simulink model "flightControlSystem"  (R2026b)
settings: Solver=ode3  StopTime=TFinal
PreLoadFcn:
  | InitVars;
  | definePX4ParamsBus;
undefined symbols (not defined in the file): control_power, DiscIntNeverNeededParam, init, MC_PITCHRATE_MAX, MC_ROLLRATE_MAX, MC_YAWRATE_MAX, PX4_Params_Default, SampleTime, timestamp
libraries: px4Utilslib x52, px4uORBlib x10, vrlib x8, aerolibutil x8, simulink x5, sharedutil x3, matrix_library x2, raspberrypiutilitieslib x2, px4Peripheralslib x2, sharedtransform x1, px4Sensorslib x1
(part 1 of 4)
settings Model: SimulationMode=external  Creator=The MathWorks, Inc.  LastModifiedBy=vishn
settings SolverCC: AutoInsertRateTranBlk=on  PositivePriorityOrder=on
settings DataIOCC: InputTimeTolerance=on
settings OptimizationCC: DifferentSizesBufferReuse=on  EfficientTunableParamExpr=on  EnhancedBackFolding=on  MaxStackSize=64  OptimizationCustomize=off  OptimizeBlockOrder=speed  PassReuseOutputArgsAs=Individual arguments  RemoveInternalMemoryZeroInit=on  RemoveRootLevelIOMemoryZeroInit=on
settings DebuggingCC: MultiTaskDSMMsg=none  ParameterPrecisionLossMsg=none  ParameterTunabilityLossMsg=error
settings HardwareCC: ProdHWDeviceType=ARM Compatible->ARM Cortex  ProdLargestAtomicFloat=Double  ProdLargestAtomicInteger=Long  ProdLongLongMode=on
settings SFSimCC: MATLABDynamicMemAlloc=off  SimTargetLang=C++
settings RTWCC: Description=Embedded Coder  HardwareBoard=PX4 Pixhawk 6c  SystemTargetFile=ert.tlc  TLCOptions="-aInlineSetEventsForThisBaseRateFcn=TLC_FALSE -aSuppressMultiTaskScheduler=TLC_FALSE  -aRateBasedStepFcn=0"  TargetLang=C++  TemplateMakefile=ert_default_tmf  Toolchain=GNU Tools for PX4 Autopilots
settings CodeAppCC: ForceParamTrailComments=on  IgnoreCustomStorageClasses=off  InsertBlockDesc=on  OperatorAnnotations=on  SFDataObjDesc=on  SimulinkDataObjDesc=on
settings ERTTargetCC: ExtModeIntrfLevel=Level2 - Open  ExtModeMexFile=ext_xcp  ExtModeStaticAlloc=on  SupportVariableSizeSignals=on

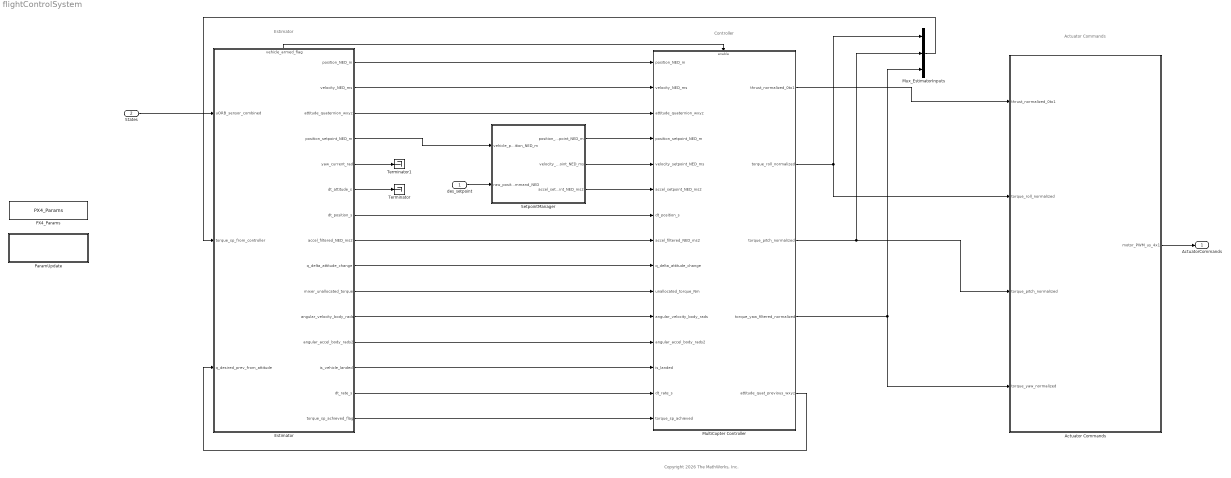
== system flightControlSystem ==
  note: Actuator Commands
  note: Estimator
  note: Controller
  note: Copyright 2026 The MathWorks, Inc.
  des_setpoint : Inport  OutDataTypeStr=Bus: desiredTargetSetpoints
  States : Inport  Port=2  OutDataTypeStr=Bus: UAVStatesBus
  Actuator Commands : Subsystem  Variant=on
  Estimator : Subsystem  Variant=on
      settings: PortSchema="{\"entries\":[{\"content\":{\"sides\":[{\"content\":{\"connectorIds\":[\"In1\",\"In2\",\"In3\"]},\"type\":\"ConnectorPlacement.EquallySpacedRectSide\",\"uuid\":\"982d90d8-ff1f-4cb9-8e33-8baf717922ad\"},{\"content\":{\"connectorIds\":[\"Out1\",\"Out2\",\"Out3\",\"Out4\",\"Out5\",\"Out6\",\"Out7\",\"Out8\",\"Out9\",\"Out10\",\"Out11\",\"Out12\",\"Out13\",\"Out14\",\"Out15\"],\"side\":\"RIGHT\"},\"type\":\"ConnectorPlacement.EquallySpacedRectSide\",\"uuid\":\"20bc02a1-8188-433b-a626-e8822f00966c\"},{\"content\":{\"connectorIds\":[\"Out16\"],\"side\":\"TOP\"},\"type\":\"ConnectorPlacement.EquallySpacedRectSide\",\"uuid\":\"edaeaf83-210e-410d-8d39-7cda3629118d\"}]},\"type\":\"ConnectorPlacement.EquallySpacedConnector\",\"uuid\":\"c0d6638f-6096-4882-ba89-b56950bc4adf\"}],\"packageUris\":[\"http://schema.mathworks.com/mf0/Connector/R2020b\"],\"version\":\"1.0\"}"
  MultiCopter Controller : Subsystem
  Mux_EstimatorInputs : Mux  Inputs=3
  PX4_Params : DataStoreMemory  DataStoreName=PX4_Params  WriteAfterWriteMsg=warning  InitialValue=PX4_Params_Default  ShowAdditionalParam=off  OutDataTypeStr=Bus: PX4_Params_Bus
  ParamUpdate : Subsystem  TreatAsAtomicUnit=on  Variant=on
  SetpointManager : Subsystem  Variant=on
  Terminator : Terminator
  Terminator1 : Terminator
  ActuatorCommands : Outport  OutDataTypeStr=Bus: setPWMInput
  wires:
  MultiCopter Controller/2(torque_roll_normalized) -> Actuator Commands/2(torque_roll_normalized), Mux_EstimatorInputs/1
  MultiCopter Controller/1(thrust_normalized_0to1) -> Actuator Commands/1(thrust_normalized_0to1)
  Estimator/11(angular_velocity_body_rads) -> MultiCopter Controller/11(angular_velocity_body_rads)
  MultiCopter Controller/4(torque_yaw_filtered_normalized) -> Mux_EstimatorInputs/3, Actuator Commands/4(torque_yaw_normalized)
  Estimator/3(attitude_quaternion_wxyz) -> MultiCopter Controller/3(attitude_quaternion_wxyz)
  MultiCopter Controller/5(attitude_quat_previous_wxyz) -> Estimator/3(q_desired_prev_from_attitude)
  SetpointManager/3(accel_setpoint_NED_ms2) -> MultiCopter Controller/6(accel_setpoint_NED_ms2)
  MultiCopter Controller/3(torque_pitch_normalized) -> Actuator Commands/3(torque_pitch_normalized), Mux_EstimatorInputs/2
  Estimator/10(mixer_unallocated_torque) -> MultiCopter Controller/10(unallocated_torque_Nm)
  Estimator/12(angular_accel_body_rads2) -> MultiCopter Controller/12(angular_accel_body_rads2)
  Mux_EstimatorInputs/1 -> Estimator/2(torque_sp_from_controller)
  Estimator/7(dt_position_s) -> MultiCopter Controller/7(dt_position_s)
  SetpointManager/1(position_setpoint_NED_m) -> MultiCopter Controller/4(position_setpoint_NED_m)
  Estimator/2(velocity_NED_ms) -> MultiCopter Controller/2(velocity_NED_ms)
  Estimator/8(accel_filtered_NED_ms2) -> MultiCopter Controller/8(accel_filtered_NED_ms2)
  Estimator/5(yaw_current_rad) -> Terminator1/1
  Estimator/6(dt_attitude_s) -> Terminator/1
  States/1 -> Estimator/1(uORB_sensor_combined)
  Actuator Commands/1(motor_PWM_us_4x1) -> ActuatorCommands/1
  Estimator/13(is_vehicle_landed) -> MultiCopter Controller/13(is_landed)
  SetpointManager/2(velocity_setpoint_NED_ms) -> MultiCopter Controller/5(velocity_setpoint_NED_ms)
  Estimator/4(position_setpoint_NED_m) -> SetpointManager/1(vehicle_position_NED_m)
  Estimator/1(position_NED_m) -> MultiCopter Controller/1(position_NED_m)
  Estimator/9(q_delta_attitude_change) -> MultiCopter Controller/9(q_delta_attitude_change)
  Estimator/16(vehicle_armed_flag) -> MultiCopter Controller/Enable
  Estimator/14(dt_rate_s) -> MultiCopter Controller/14(dt_rate_s)
  Estimator/15(torque_sp_achieved_flag) -> MultiCopter Controller/15(torque_sp_achieved)
  des_setpoint/1 -> SetpointManager/2(raw_position_command_NED)

== system flightControlSystem/Actuator Commands ==
  note: Simulation = true:
      | The subsystem processes the tau and thrust signals, computes the multicopter mixers, and generates the PWM signals required by the plant for closed-loop simulation.
      |
      | Simulation = false:
      | The subsystem processes the tau and thrust signals output from the controller and publishes them to the Torque and Thrust block. The PX4 mixer then computes the required outputs based on the selected multicopter configuration for flight operations.
  thrust_normalized_0to1 : Inport
  torque_roll_normalized : Inport  Port=2
  torque_pitch_normalized : Inport  Port=3
  torque_yaw_normalized : Inport  Port=4
  Actuator Commands : Subsystem  VariantControl=Simulation == false
  Simulation Actuator Commands : Subsystem  VariantControl=Simulation == true
  motor_PWM_us_4x1 : Outport

== system flightControlSystem/Estimator ==
  note: Simulation = true:
      | The subsystem provides the required estimator values from the 6-DoF Dynamics feedback for closed-loop simulation with the controller.
      |
      | Simulation = false:
      | The subsystem reads the required PX4 estimator values for the flight controller from the uOrb block.
  uORB_sensor_combined : Inport
  torque_sp_from_controller : Inport  Port=2
  q_desired_prev_from_attitude : Inport  Port=3
  Estimator : Subsystem  VariantControl=Simulation == false
  Simulation Estimator : Subsystem  VariantControl=Simulation == true
  position_NED_m : Outport
  velocity_NED_ms : Outport  Port=2
  attitude_quaternion_wxyz : Outport  Port=3
  position_setpoint_NED_m : Outport  Port=4
  yaw_current_rad : Outport  Port=5
  dt_attitude_s : Outport  Port=6
  dt_position_s : Outport  Port=7
  accel_filtered_NED_ms2 : Outport  Port=8
  q_delta_attitude_change : Outport  Port=9
  mixer_unallocated_torque : Outport  Port=10
  angular_velocity_body_rads : Outport  Port=11
  angular_accel_body_rads2 : Outport  Port=12
  is_vehicle_landed : Outport  Port=13
  dt_rate_s : Outport  Port=14
  torque_sp_achieved_flag : Outport  Port=15
  vehicle_armed_flag : Outport  Port=16

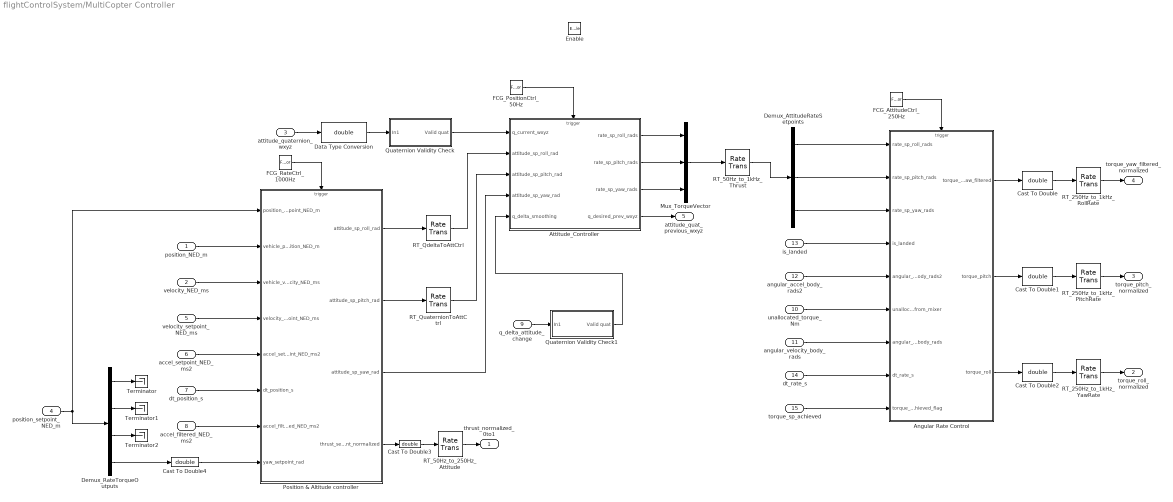
== system flightControlSystem/MultiCopter Controller ==
  position_NED_m : Inport
  velocity_NED_ms : Inport  Port=2
  attitude_quaternion_wxyz : Inport  Port=3
  position_setpoint_NED_m : Inport  Port=4
  velocity_setpoint_NED_ms : Inport  Port=5
  accel_setpoint_NED_ms2 : Inport  Port=6
  dt_position_s : Inport  Port=7
  accel_filtered_NED_ms2 : Inport  Port=8
  q_delta_attitude_change : Inport  Port=9
  unallocated_torque_Nm : Inport  Port=10
  angular_velocity_body_rads : Inport  Port=11
  angular_accel_body_rads2 : Inport  Port=12
  is_landed : Inport  Port=13
  dt_rate_s : Inport  Port=14
  torque_sp_achieved : Inport  Port=15
  Enable : EnablePort
  Angular Rate Control : Subsystem
  Attitude_Controller : Subsystem
  Cast To Double{,1..4} (5 alike) : DataTypeConversion  OutDataTypeStr=double  SaturateOnIntegerOverflow=off  RndMeth=Floor
  Data Type Conversion : DataTypeConversion  OutDataTypeStr=double  SaturateOnIntegerOverflow=off  RndMeth=Floor
  Demux_AttitudeRateSetpoints : Demux  Outputs=3
  Demux_RateTorqueOutputs : Demux
  FCG_AttitudeCtrl_250Hz : FunctionCallGenerator  SampleTime=0.001
  FCG_PositionCtrl_50Hz : FunctionCallGenerator  SampleTime=0.004
  FCG_RateCtrl_1000Hz : FunctionCallGenerator  SampleTime=0.02
  Mux_TorqueVector : Mux  Inputs=3
  Position & Altitude controller : Subsystem
  Quaternion Validity Check : Subsystem
  Quaternion Validity Check1 : Subsystem
  RT_250Hz_to_1kHz_PitchRate : RateTransition  OutPortSampleTime=SampleTime
  RT_250Hz_to_1kHz_RollRate : RateTransition  OutPortSampleTime=SampleTime
  RT_250Hz_to_1kHz_YawRate : RateTransition  OutPortSampleTime=SampleTime
  RT_50Hz_to_1kHz_Thrust : RateTransition
  RT_50Hz_to_250Hz_Attitude : RateTransition  OutPortSampleTime=SampleTime
  RT_QdeltaToAttCtrl : RateTransition
  RT_QuaternionToAttCtrl : RateTransition
  Terminator : Terminator
  Terminator1 : Terminator
  Terminator2 : Terminator
  thrust_normalized_0to1 : Outport
  torque_roll_normalized : Outport  Port=2
  torque_pitch_normalized : Outport  Port=3
  torque_yaw_filtered_normalized : Outport  Port=4
  attitude_quat_previous_wxyz : Outport  Port=5
  wires:
  unallocated_torque_Nm/1 -> Angular Rate Control/6(unallocated_torque_from_mixer)
  Demux_RateTorqueOutputs/4 -> Cast To Double4/1
  Demux_RateTorqueOutputs/2 -> Terminator1/1
  Demux_RateTorqueOutputs/3 -> Terminator2/1
  Data Type Conversion/1 -> Quaternion Validity Check/1(In1)
  attitude_quaternion_wxyz/1 -> Data Type Conversion/1
  Quaternion Validity Check/1(Valid quat) -> Attitude_Controller/1(q_current_wxyz)
  position_setpoint_NED_m/1 -> Position & Altitude controller/1(position_setpoint_NED_m), Demux_RateTorqueOutputs/1
  Demux_RateTorqueOutputs/1 -> Terminator/1
  q_delta_attitude_change/1 -> Quaternion Validity Check1/1(In1)
  FCG_RateCtrl_1000Hz/1 -> Position & Altitude controller/Trigger
  Attitude_Controller/4(q_desired_prev_wxyz) -> attitude_quat_previous_wxyz/1
  position_NED_m/1 -> Position & Altitude controller/2(vehicle_position_NED_m)
  dt_rate_s/1 -> Angular Rate Control/8(dt_rate_s)
  velocity_NED_ms/1 -> Position & Altitude controller/3(vehicle_velocity_NED_ms)
  angular_accel_body_rads2/1 -> Angular Rate Control/5(angular_accel_body_rads2)
  velocity_setpoint_NED_ms/1 -> Position & Altitude controller/4(velocity_setpoint_NED_ms)
  RT_250Hz_to_1kHz_YawRate/1 -> torque_roll_normalized/1
  Angular Rate Control/3(torque_roll) -> Cast To Double2/1
  Cast To Double4/1 -> Position & Altitude controller/8(yaw_setpoint_rad)
  accel_setpoint_NED_ms2/1 -> Position & Altitude controller/5(accel_setpoint_NED_ms2)
  dt_position_s/1 -> Position & Altitude controller/6(dt_position_s)
  RT_250Hz_to_1kHz_RollRate/1 -> torque_yaw_filtered_normalized/1
  Quaternion Validity Check1/1(Valid quat) -> Attitude_Controller/5(q_delta_smoothing)
  accel_filtered_NED_ms2/1 -> Position & Altitude controller/7(accel_filtered_NED_ms2)
  Position & Altitude controller/2(attitude_sp_pitch_rad) -> RT_QuaternionToAttCtrl/1
  Position & Altitude controller/3(attitude_sp_yaw_rad) -> Attitude_Controller/4(attitude_sp_yaw_rad)
  Position & Altitude controller/1(attitude_sp_roll_rad) -> RT_QdeltaToAttCtrl/1
  Position & Altitude controller/4(thrust_setpoint_normalized) -> Cast To Double3/1
  FCG_PositionCtrl_50Hz/1 -> Attitude_Controller/Trigger
  RT_QdeltaToAttCtrl/1 -> Attitude_Controller/2(attitude_sp_roll_rad)
  RT_QuaternionToAttCtrl/1 -> Attitude_Controller/3(attitude_sp_pitch_rad)
  Cast To Double3/1 -> RT_50Hz_to_250Hz_Attitude/1
  RT_50Hz_to_1kHz_Thrust/1 -> Demux_AttitudeRateSetpoints/1
  is_landed/1 -> Angular Rate Control/4(is_landed)
  RT_50Hz_to_250Hz_Attitude/1 -> thrust_normalized_0to1/1
  Mux_TorqueVector/1 -> RT_50Hz_to_1kHz_Thrust/1
  FCG_AttitudeCtrl_250Hz/1 -> Angular Rate Control/Trigger
  RT_250Hz_to_1kHz_PitchRate/1 -> torque_pitch_normalized/1
  angular_velocity_body_rads/1 -> Angular Rate Control/7(angular_velocity_body_rads)
  torque_sp_achieved/1 -> Angular Rate Control/9(torque_sp_achieved_flag)
  Angular Rate Control/1(torque_yaw_filtered) -> Cast To Double/1
  Angular Rate Control/2(torque_pitch) -> Cast To Double1/1
  Cast To Double1/1 -> RT_250Hz_to_1kHz_PitchRate/1
  Cast To Double/1 -> RT_250Hz_to_1kHz_RollRate/1
  Cast To Double2/1 -> RT_250Hz_to_1kHz_YawRate/1
  Attitude_Controller/1(rate_sp_roll_rads) -> Mux_TorqueVector/1
  Attitude_Controller/2(rate_sp_pitch_rads) -> Mux_TorqueVector/2
  Attitude_Controller/3(rate_sp_yaw_rads) -> Mux_TorqueVector/3
  Demux_AttitudeRateSetpoints/1 -> Angular Rate Control/1(rate_sp_roll_rads)
  Demux_AttitudeRateSetpoints/2 -> Angular Rate Control/2(rate_sp_pitch_rads)
  Demux_AttitudeRateSetpoints/3 -> Angular Rate Control/3(rate_sp_yaw_rads)

== system flightControlSystem/ParamUpdate ==
  note: 1) Add Subsystem or Model blocks as valid variant choices.
      | 2) You cannot connect blocks at this level. At simulation, connectivity is automatically
      | determined, based on the active variant and port name matching.
  HW_ParamUpdate : Subsystem  VariantControl=Simulation == false
  SimParamUpdate : Subsystem  VariantControl=Simulation == true

== system flightControlSystem/SetpointManager ==
  note: Simulation = true:
      | The subsystem forwards the target setpoint signal from the PerceptionGuidance block as a bus signal for controller processing.
      |
      | Simulation = false:
      | The subsystem reads the target setpoint values from the Serial Read block and makes them available to the flight controller.
  vehicle_position_NED_m : Inport
  raw_position_command_NED : Inport  Port=2
  Set target Position : Subsystem  VariantControl=Simulation == false
  Simulation Set target Position : Subsystem  VariantControl=Simulation == true
  position_setpoint_NED_m : Outport
  velocity_setpoint_NED_ms : Outport  Port=2
  accel_setpoint_NED_ms2 : Outport  Port=3

== system flightControlSystem/Actuator Commands/Actuator Commands ==
  thrust_normalized_0to1 : Inport
  torque_pitch_normalized : Inport  Port=2
  torque_roll_normalized : Inport  Port=3
  torque_yaw_normalized : Inport  Port=4
  Bus Creator1 : BusCreator  Inputs=8  OutDataTypeStr=Bus: setPWMInput
  Demux2 : Demux  Outputs=8
  MATLAB Function : MATLAB Function  TreatAsAtomicUnit=on
  "Using PX4 Mixers " : Subsystem  VariantControl=isUsingSimulinkMixer==false
  motor_PWM_us_4x1 : Outport
  wires:
  MATLAB Function/1(y) -> Demux2/1
  thrust_normalized_0to1/1 -> "Using PX4 Mixers "/1(tau_Thrust)
  torque_pitch_normalized/1 -> "Using PX4 Mixers "/2(tau_Pitch)
  torque_roll_normalized/1 -> "Using PX4 Mixers "/3(tau_Roll)
  Demux2/7 -> Bus Creator1/7  "M7"
  Demux2/5 -> Bus Creator1/5  "M5"
  Demux2/1 -> Bus Creator1/1  "M1"
  Demux2/3 -> Bus Creator1/3  "M3"
  Demux2/8 -> Bus Creator1/8  "M8"
  Demux2/6 -> Bus Creator1/6  "M6"
  Demux2/4 -> Bus Creator1/4  "M4"
  Demux2/2 -> Bus Creator1/2  "M2"
  torque_yaw_normalized/1 -> "Using PX4 Mixers "/4(tau_yaw)
  Bus Creator1/1 -> motor_PWM_us_4x1/1

== system flightControlSystem/Actuator Commands/Simulation Actuator Commands ==
  thrust_normalized_0to1 : Inport
  torque_pitch_normalized : Inport  Port=2
  torque_roll_normalized : Inport  Port=3
  torque_yaw_normalized : Inport  Port=4
  Mixer : Subsystem
  motor_PWM_us_4x1 : Outport
  wires:
  thrust_normalized_0to1/1 -> Mixer/1(tau_Thrust)
  Mixer/1(PWM_Input) -> motor_PWM_us_4x1/1
  torque_yaw_normalized/1 -> Mixer/2(tau_yaw)
  torque_pitch_normalized/1 -> Mixer/3(tau_Pitch)
  torque_roll_normalized/1 -> Mixer/4(tau_Roll)

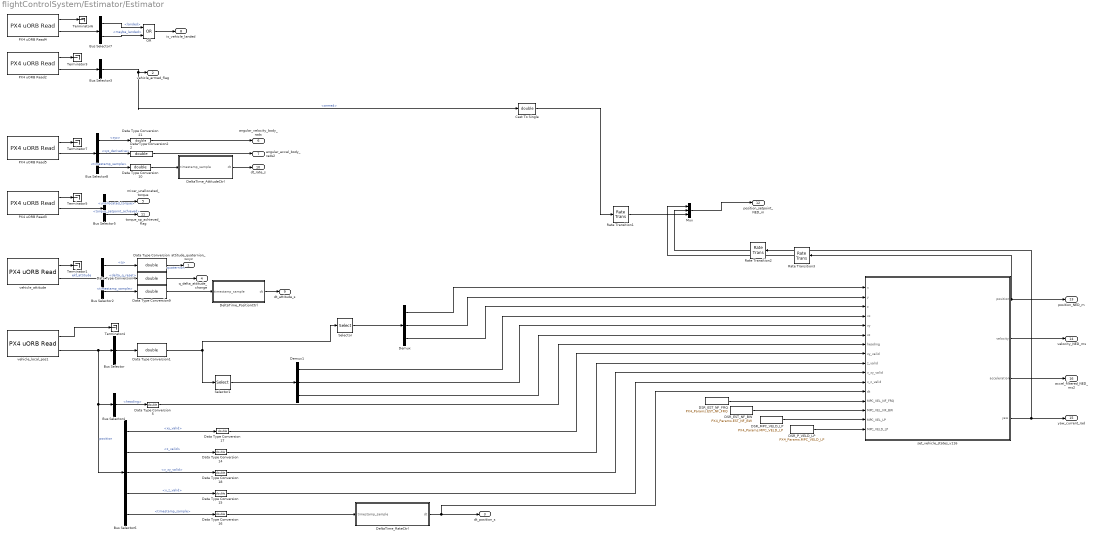
== system flightControlSystem/Estimator/Estimator ==
  Bus Selector : BusSelector  OutputSignals=x,y,z,vx,vy,vz,heading  OutputAsBus=on
  Bus Selector2 : BusSelector  OutputSignals=q,delta_q_reset,timestamp_sample
  Bus Selector3 : BusSelector  OutputSignals=armed
  Bus Selector4 : BusSelector  OutputSignals=heading
  Bus Selector5 : BusSelector  OutputSignals=unallocated_torque,torque_setpoint_achieved
  Bus Selector6 : BusSelector  OutputSignals=xy_valid,z_valid,v_xy_valid,v_z_valid,timestamp_sample
  Bus Selector7 : BusSelector  OutputSignals=landed,maybe_landed
  Bus Selector8 : BusSelector  OutputSignals=xyz,xyz_derivative,timestamp_sample
  Cast To Single : DataTypeConversion  OutDataTypeStr=double  SaturateOnIntegerOverflow=off  RndMeth=Floor
  DSR_EST_NF_BW : DataStoreRead  DataStoreName=PX4_Params  DataStoreElements=PX4_Params.EST_NF_BW  IndexOptions=Index vector (dialog)  Indices=1  OutputSizes=1
  DSR_EST_NF_FRQ : DataStoreRead  DataStoreName=PX4_Params  DataStoreElements=PX4_Params.EST_NF_FRQ  IndexOptions=Index vector (dialog)  Indices=1  OutputSizes=1
  DSR_MPC_VELD_LP : DataStoreRead  DataStoreName=PX4_Params  DataStoreElements=PX4_Params.MPC_VELD_LP  IndexOptions=Index vector (dialog)  Indices=1  OutputSizes=1
  DSR_P_VELD_LP : DataStoreRead  DataStoreName=PX4_Params  DataStoreElements=PX4_Params.MPC_VELD_LP  IndexOptions=Index vector (dialog)  Indices=1  OutputSizes=1
  Data Type Conversion{,1,4..5,9..10,14..18,21..22} (13 alike) : DataTypeConversion  OutDataTypeStr=double  SaturateOnIntegerOverflow=off  RndMeth=Floor
  DeltaTime_AttitudeCtrl : MATLAB Function  TreatAsAtomicUnit=on
  DeltaTime_PositionCtrl : MATLAB Function  TreatAsAtomicUnit=on
  DeltaTime_RateCtrl : MATLAB Function  TreatAsAtomicUnit=on
  Demux : Demux  Outputs=3
  Demux1 : Demux  Outputs=3
  Mux : Mux  Inputs=3
  OR : Logic  Operator=OR  IconShape=distinctive  AllPortsSameDT=off  OutDataTypeStr=boolean
  PX4 uORB Read2 : px4uORBlib/PX4 uORB Read  uORBMsg=ActuatorArmed  uORBTopicName=actuator_armed  SubscribeNonZeroInstance=off  selectInstanceNum=1  SampleTime=-1  isSingleTopicMsg=on  BlockingMode=off  BlockTimeout=1e-3
  PX4 uORB Read3 : px4uORBlib/PX4 uORB Read  uORBMsg=ControlAllocatorStatus  uORBTopicName=control_allocator_status  SubscribeNonZeroInstance=off  selectInstanceNum=1  SampleTime=-1  isSingleTopicMsg=on  BlockingMode=off  BlockTimeout=1e-3
  PX4 uORB Read4 : px4uORBlib/PX4 uORB Read  uORBMsg=VehicleLandDetected  uORBTopicName=vehicle_land_detected  SubscribeNonZeroInstance=off  selectInstanceNum=1  SampleTime=-1  isSingleTopicMsg=on  BlockingMode=off  BlockTimeout=1e-3
  PX4 uORB Read5 : px4uORBlib/PX4 uORB Read  uORBMsg=VehicleAngularVelocity  uORBTopicName=vehicle_angular_velocity  SubscribeNonZeroInstance=off  selectInstanceNum=1  SampleTime=-1  isSingleTopicMsg=off  BlockingMode=off  BlockTimeout=1e-3
  Rate Transition1 : RateTransition
  Rate Transition2 : RateTransition
  Rate Transition3 : RateTransition
  Selector : Selector  InputPortWidth=7  IndexOptions=Index vector (dialog)  Indices=[1:3]  OutputSizes=1  RuntimeRangeChecks=off
  Selector1 : Selector  InputPortWidth=7  IndexOptions=Index vector (dialog)  Indices=[4:6]  OutputSizes=1  RuntimeRangeChecks=off
  Terminator{1,3..7} (6 alike) : Terminator
  set_vehicle_states_v116 : MATLAB Function  TreatAsAtomicUnit=on
  vehicle_attitude : px4uORBlib/PX4 uORB Read  uORBMsg=VehicleAttitude  uORBTopicName=vehicle_attitude  SubscribeNonZeroInstance=off  selectInstanceNum=1  SampleTime=-1  isSingleTopicMsg=off  BlockingMode=off  BlockTimeout=1e-3
  vehicle_local_pos1 : px4uORBlib/PX4 uORB Read  uORBMsg=VehicleLocalPosition  uORBTopicName=vehicle_local_position  SubscribeNonZeroInstance=off  selectInstanceNum=1  SampleTime=-1  isSingleTopicMsg=off  BlockingMode=off  BlockTimeout=1e-3
  attitude_quaternion_wxyz : Outport
  vehicle_armed_flag : Outport  Port=2
  dt_position_s : Outport  Port=3
  q_delta_attitude_change : Outport  Port=4
  mixer_unallocated_torque : Outport  Port=5
  angular_velocity_body_rads : Outport  Port=6
  angular_accel_body_rads2 : Outport  Port=7
  is_vehicle_landed : Outport  Port=8
  dt_attitude_s : Outport  Port=9
  dt_rate_s : Outport  Port=10
  torque_sp_achieved_flag : Outport  Port=11
  position_setpoint_NED_m : Outport  Port=12
  position_NED_m : Outport  Port=13
  velocity_NED_ms : Outport  Port=14
  yaw_current_rad : Outport  Port=15
  accel_filtered_NED_ms2 : Outport  Port=16
  wires:
  Data Type Conversion/1 -> attitude_quaternion_wxyz/1  "quaternion"
  PX4 uORB Read2/1 -> Terminator3/1
  PX4 uORB Read3/2 -> Bus Selector5/1
  OR/1 -> is_vehicle_landed/1
  PX4 uORB Read4/2 -> Bus Selector7/1
  PX4 uORB Read3/1 -> Terminator5/1
  Data Type Conversion1/1 -> Selector/1, Selector1/1
  PX4 uORB Read2/2 -> Bus Selector3/1
  PX4 uORB Read4/1 -> Terminator6/1
  Data Type Conversion14/1 -> set_vehicle_states_v116/9(z_valid)
  Data Type Conversion10/1 -> DeltaTime_AttitudeCtrl/1(timestamp_sample)
  PX4 uORB Read5/2 -> Bus Selector8/1
  Selector/1 -> Demux/1
  PX4 uORB Read5/1 -> Terminator7/1
  Data Type Conversion18/1 -> set_vehicle_states_v116/10(v_xy_valid)
  vehicle_attitude/1 -> Terminator1/1
  Data Type Conversion15/1 -> set_vehicle_states_v116/11(v_z_valid)
  vehicle_attitude/2 -> Bus Selector2/1  "ekf_attitude"
  Data Type Conversion22/1 -> angular_accel_body_rads2/1
  vehicle_local_pos1/1 -> Terminator4/1
  Data Type Conversion4/1 -> q_delta_attitude_change/1
  vehicle_local_pos1/2 -> Bus Selector/1, Bus Selector4/1, Bus Selector6/1  "position"
  Bus Selector8/1 -> Data Type Conversion21/1  "<xyz>"
  Bus Selector7/1 -> OR/1  "<landed>"
  Bus Selector8/2 -> Data Type Conversion22/1  "<xyz_derivative>"
  Bus Selector7/2 -> OR/2  "<maybe_landed>"
  Demux1/1 -> set_vehicle_states_v116/4(vx)
  Demux/2 -> set_vehicle_states_v116/2(y)
  Data Type Conversion9/1 -> DeltaTime_PositionCtrl/1(timestamp_sample)
  Bus Selector2/2 -> Data Type Conversion4/1  "<delta_q_reset>"
  Bus Selector3/1 -> Cast To Single/1, vehicle_armed_flag/1  "<armed>"
  Bus Selector8/3 -> Data Type Conversion10/1  "<timestamp_sample>"
  Bus Selector6/2 -> Data Type Conversion14/1  "<z_valid>"
  Bus Selector5/1 -> mixer_unallocated_torque/1  "<unallocated_torque>"
  Bus Selector6/4 -> Data Type Conversion15/1  "<v_z_valid>"
  Bus Selector5/2 -> torque_sp_achieved_flag/1  "<torque_setpoint_achieved>"
  Demux/1 -> set_vehicle_states_v116/1(x)
  Bus Selector4/1 -> Data Type Conversion5/1  "<heading>"
  Bus Selector2/1 -> Data Type Conversion/1  "<q>"
  Demux1/2 -> set_vehicle_states_v116/5(vy)
  Demux/3 -> set_vehicle_states_v116/3(z)
  Bus Selector2/3 -> Data Type Conversion9/1  "<timestamp_sample>"
  Bus Selector/1 -> Data Type Conversion1/1
  Data Type Conversion16/1 -> DeltaTime_RateCtrl/1(timestamp_sample)
  Data Type Conversion21/1 -> angular_velocity_body_rads/1
  Data Type Conversion5/1 -> set_vehicle_states_v116/7(heading)
  Bus Selector6/5 -> Data Type Conversion16/1  "<timestamp_sample>"
  Bus Selector6/1 -> Data Type Conversion17/1  "<xy_valid>"
  Bus Selector6/3 -> Data Type Conversion18/1  "<v_xy_valid>"
  DeltaTime_AttitudeCtrl/1(dt) -> dt_rate_s/1
  DeltaTime_PositionCtrl/1(dt) -> dt_attitude_s/1
  Selector1/1 -> Demux1/1
  Data Type Conversion17/1 -> set_vehicle_states_v116/8(xy_valid)
  Demux1/3 -> set_vehicle_states_v116/6(vz)
  DeltaTime_RateCtrl/1(dt) -> set_vehicle_states_v116/12(dt), dt_position_s/1
  Rate Transition1/1 -> Mux/3
  Mux/1 -> position_setpoint_NED_m/1
  DSR_EST_NF_FRQ/1 -> set_vehicle_states_v116/13(MPC_VEL_NF_FRQ)
  DSR_EST_NF_BW/1 -> set_vehicle_states_v116/14(MPC_VEL_NF_BW)
  DSR_MPC_VELD_LP/1 -> set_vehicle_states_v116/15(MPC_VEL_LP)
  DSR_P_VELD_LP/1 -> set_vehicle_states_v116/16(MPC_VELD_LP)
  set_vehicle_states_v116/1(position) -> position_NED_m/1, Rate Transition3/1
  set_vehicle_states_v116/2(velocity) -> velocity_NED_ms/1
  set_vehicle_states_v116/3(acceleration) -> accel_filtered_NED_ms2/1
  set_vehicle_states_v116/4(yaw) -> Rate Transition2/1, yaw_current_rad/1
  Rate Transition2/1 -> Mux/2
  Rate Transition3/1 -> Mux/1
  Cast To Single/1 -> Rate Transition1/1

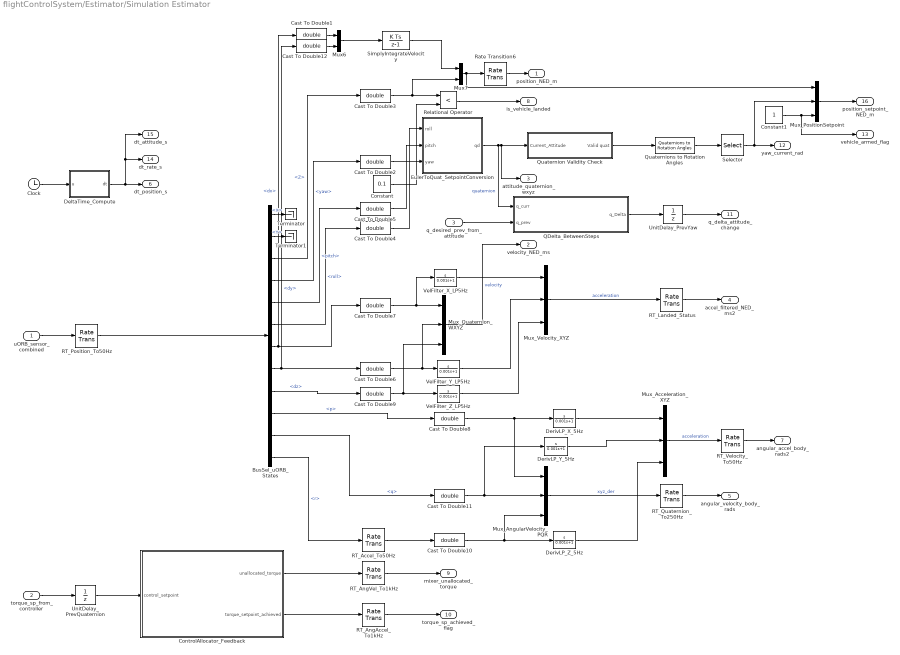
== system flightControlSystem/Estimator/Simulation Estimator ==
  uORB_sensor_combined : Inport
  torque_sp_from_controller : Inport  Port=2
  q_desired_prev_from_attitude : Inport  Port=3
  BusSel_uORB_States : BusSelector  OutputSignals=X,Y,Z,yaw,pitch,roll,dx,dy,dz,p,q,r
  Cast To Double{1..12} (12 alike) : DataTypeConversion  OutDataTypeStr=double  SaturateOnIntegerOverflow=off  RndMeth=Floor
  Clock : Clock
  Constant : Constant  Value=0.1  SampleTime=-1
  Constant1 : Constant  SampleTime=-1
  ControlAllocator_Feedback : MATLAB Function  TreatAsAtomicUnit=on
  DeltaTime_Compute : MATLAB Function  TreatAsAtomicUnit=on
  DerivLP_X_5Hz : TransferFcn  Numerator=[1 0]  Denominator=[0.001 1]
  DerivLP_Y_5Hz : TransferFcn  Numerator=[1 0]  Denominator=[0.001 1]
  DerivLP_Z_5Hz : TransferFcn  Numerator=[1 0]  Denominator=[0.001 1]
  EulerToQuat_SetpointConversion : MATLAB Function  TreatAsAtomicUnit=on
  Mux6 : Mux  Inputs=2
  Mux7 : Mux  Inputs=2
  Mux_Acceleration_XYZ : Mux  Inputs=3
  Mux_AngularVelocity_PQR : Mux  Inputs=3
  Mux_PositionSetpoint : Mux  Inputs=3
  Mux_Quaternion_WXYZ : Mux  Inputs=3
  Mux_Velocity_XYZ : Mux  Inputs=3
  QDelta_BetweenSteps : MATLAB Function  TreatAsAtomicUnit=on
  Quaternion Validity Check : Subsystem
  Quaternions to Rotation Angles : sharedtransform/Quaternions to Rotation Angles  rotationOrder=ZYX  aMode=aMode
  RT_Accel_To50Hz : RateTransition  OutPortSampleTime=SampleTime
  RT_AngAccel_To1kHz : RateTransition
  RT_AngVel_To1kHz : RateTransition
  RT_Landed_Status : RateTransition
  RT_Position_To50Hz : RateTransition  OutPortSampleTime=SampleTime
  RT_Quaternion_To250Hz : RateTransition
  RT_Velocity_To50Hz : RateTransition
  Rate Transition6 : RateTransition
  Relational Operator : RelationalOperator  Operator=<  OutDataTypeStr=boolean  RndMeth=Simplest  InputSameDT=off
  Selector : Selector  InputPortWidth=3  IndexOptions=Index vector (dialog)  Indices=1  OutputSizes=1  RuntimeRangeChecks=off
  SimplyIntegrateVelocity : DiscreteIntegrator  InitialCondition=init.posNED(1:2)  SampleTime=0.005  ICPrevOutput=DiscIntNeverNeededParam  ICPrevScaledInput=DiscIntNeverNeededParam
  Terminator : Terminator
  Terminator1 : Terminator
  UnitDelay_PrevQuaternion : UnitDelay  InitialCondition=[0,0,0]  SampleTime=-1
  UnitDelay_PrevYaw : UnitDelay  InitialCondition=[1,0,0,0]  SampleTime=-1
  VelFilter_X_LP5Hz : TransferFcn  Numerator=[1 0]  Denominator=[0.001 1]
  VelFilter_Y_LP5Hz : TransferFcn  Numerator=[1 0]  Denominator=[0.001 1]
  VelFilter_Z_LP5Hz : TransferFcn  Numerator=[1 0]  Denominator=[0.001 1]
  position_NED_m : Outport
  velocity_NED_ms : Outport  Port=2
  attitude_quaternion_wxyz : Outport  Port=3
  accel_filtered_NED_ms2 : Outport  Port=4
  angular_velocity_body_rads : Outport  Port=5
  dt_position_s : Outport  Port=6
  angular_accel_body_rads2 : Outport  Port=7
  is_vehicle_landed : Outport  Port=8
  mixer_unallocated_torque : Outport  Port=9
  torque_sp_achieved_flag : Outport  Port=10
  q_delta_attitude_change : Outport  Port=11
  yaw_current_rad : Outport  Port=12
  vehicle_armed_flag : Outport  Port=13
  dt_rate_s : Outport  Port=14
  dt_attitude_s : Outport  Port=15
  position_setpoint_NED_m : Outport  Port=16
  wires:
  Quaternions to Rotation Angles/1 -> Selector/1
  uORB_sensor_combined/1 -> RT_Position_To50Hz/1
  Clock/1 -> DeltaTime_Compute/1(u)
  Selector/1 -> Mux_PositionSetpoint/2, yaw_current_rad/1
  Constant1/1 -> Mux_PositionSetpoint/3, vehicle_armed_flag/1
  RT_Velocity_To50Hz/1 -> angular_accel_body_rads2/1
  VelFilter_X_LP5Hz/1 -> Mux_Velocity_XYZ/1
  torque_sp_from_controller/1 -> UnitDelay_PrevQuaternion/1
  Cast To Double2/1 -> EulerToQuat_SetpointConversion/3(yaw)
  UnitDelay_PrevQuaternion/1 -> ControlAllocator_Feedback/1(control_setpoint)
  RT_Position_To50Hz/1 -> BusSel_uORB_States/1
  RT_AngVel_To1kHz/1 -> mixer_unallocated_torque/1
  BusSel_uORB_States/11 -> Cast To Double11/1  "<q>"
  DeltaTime_Compute/1(dt) -> dt_rate_s/1, dt_attitude_s/1, dt_position_s/1
  Cast To Double4/1 -> EulerToQuat_SetpointConversion/1(roll)
  DerivLP_Y_5Hz/1 -> Mux_Acceleration_XYZ/2
  BusSel_uORB_States/3 -> Cast To Double3/1  "<Z>"
  Cast To Double5/1 -> EulerToQuat_SetpointConversion/2(pitch)
  BusSel_uORB_States/4 -> Cast To Double2/1  "<yaw>"
  DerivLP_X_5Hz/1 -> Mux_Acceleration_XYZ/1
  BusSel_uORB_States/5 -> Cast To Double5/1  "<pitch>"
  RT_Quaternion_To250Hz/1 -> angular_velocity_body_rads/1
  BusSel_uORB_States/6 -> Cast To Double4/1  "<roll>"
  Cast To Double6/1 -> Mux_Quaternion_WXYZ/2, VelFilter_Y_LP5Hz/1
  BusSel_uORB_States/7 -> Cast To Double7/1, Cast To Double1/1  "<dx>"
  DerivLP_Z_5Hz/1 -> Mux_Acceleration_XYZ/3
  RT_AngAccel_To1kHz/1 -> torque_sp_achieved_flag/1
  BusSel_uORB_States/8 -> Cast To Double6/1, Cast To Double12/1  "<dy>"
  RT_Accel_To50Hz/1 -> Cast To Double10/1
  BusSel_uORB_States/9 -> Cast To Double9/1  "<dz>"
  Cast To Double7/1 -> VelFilter_X_LP5Hz/1, Mux_Quaternion_WXYZ/1
  BusSel_uORB_States/10 -> Cast To Double8/1  "<p>"
  BusSel_uORB_States/12 -> RT_Accel_To50Hz/1  "<r>"
  ControlAllocator_Feedback/1(unallocated_torque) -> RT_AngVel_To1kHz/1
  ControlAllocator_Feedback/2(torque_setpoint_achieved) -> RT_AngAccel_To1kHz/1
  q_desired_prev_from_attitude/1 -> QDelta_BetweenSteps/2(q_prev)
  Cast To Double3/1 -> Mux7/2, Relational Operator/1
  Constant/1 -> Relational Operator/2
  Cast To Double9/1 -> VelFilter_Z_LP5Hz/1, Mux_Quaternion_WXYZ/3
  VelFilter_Y_LP5Hz/1 -> Mux_Velocity_XYZ/2
  Relational Operator/1 -> is_vehicle_landed/1
  EulerToQuat_SetpointConversion/1(qd) -> attitude_quaternion_wxyz/1, Quaternion Validity Check/1(Current_Attitude), QDelta_BetweenSteps/1(q_curr)  "quaternion"
  Mux_Quaternion_WXYZ/1 -> velocity_NED_ms/1  "velocity"
  VelFilter_Z_LP5Hz/1 -> Mux_Velocity_XYZ/3
  Cast To Double8/1 -> DerivLP_X_5Hz/1, Mux_AngularVelocity_PQR/1
  UnitDelay_PrevYaw/1 -> q_delta_attitude_change/1
  Cast To Double11/1 -> DerivLP_Y_5Hz/1, Mux_AngularVelocity_PQR/2
  RT_Landed_Status/1 -> accel_filtered_NED_ms2/1
  Cast To Double10/1 -> DerivLP_Z_5Hz/1, Mux_AngularVelocity_PQR/3
  Quaternion Validity Check/1(Valid quat) -> Quaternions to Rotation Angles/1
  Mux_Velocity_XYZ/1 -> RT_Landed_Status/1  "acceleration"
  QDelta_BetweenSteps/1(q_Delta) -> UnitDelay_PrevYaw/1
  Mux_AngularVelocity_PQR/1 -> RT_Quaternion_To250Hz/1  "xyz_der"
  Mux_Acceleration_XYZ/1 -> RT_Velocity_To50Hz/1  "acceleration"
  Mux_PositionSetpoint/1 -> position_setpoint_NED_m/1
  Rate Transition6/1 -> position_NED_m/1
  Mux6/1 -> SimplyIntegrateVelocity/1
  Mux7/1 -> Mux_PositionSetpoint/1, Rate Transition6/1
  SimplyIntegrateVelocity/1 -> Mux7/1
  Cast To Double1/1 -> Mux6/1
  Cast To Double12/1 -> Mux6/2
  BusSel_uORB_States/1 -> Terminator/1  "<X>"
  BusSel_uORB_States/2 -> Terminator1/1  "<Y>"

== system flightControlSystem/MultiCopter Controller/Angular Rate Control ==
  rate_sp_roll_rads : Inport
  rate_sp_pitch_rads : Inport  Port=2
  rate_sp_yaw_rads : Inport  Port=3
  is_landed : Inport  Port=4
  angular_accel_body_rads2 : Inport  Port=5
  unallocated_torque_from_mixer : Inport  Port=6
  angular_velocity_body_rads : Inport  Port=7
  dt_rate_s : Inport  Port=8
  torque_sp_achieved_flag : Inport  Port=9
  function : TriggerPort  TriggerType=function-call  VariantControl=(inherit)
  Cast To Double : DataTypeConversion  OutDataTypeStr=double  SaturateOnIntegerOverflow=off  RndMeth=Floor
  Cast To Single : DataTypeConversion  OutDataTypeStr=single  SaturateOnIntegerOverflow=off  RndMeth=Floor
  ControlPower_Monitor : MATLAB Function  TreatAsAtomicUnit=on
  DSR_IntegratorLimits : DataStoreRead  DataStoreName=PX4_Params  DataStoreElements=PX4_Params.MC_RATE_INT_LIM  IndexOptions=Index vector (dialog)  Indices=1  OutputSizes=1
  DSR_MC_RATE_D_Gains : DataStoreRead  DataStoreName=PX4_Params  DataStoreElements=PX4_Params.MC_RATE_D  IndexOptions=Index vector (dialog)  Indices=1  OutputSizes=1
  DSR_MC_RATE_FF_Gains : DataStoreRead  DataStoreName=PX4_Params  DataStoreElements=PX4_Params.MC_RATE_FF  IndexOptions=Index vector (dialog)  Indices=1  OutputSizes=1
  DSR_MC_RATE_I_Gains : DataStoreRead  DataStoreName=PX4_Params  DataStoreElements=PX4_Params.MC_RATE_I  IndexOptions=Index vector (dialog)  Indices=1  OutputSizes=1
  DSR_MC_RATE_P_Gains : DataStoreRead  DataStoreName=PX4_Params  DataStoreElements=PX4_Params.MC_RATE_P  IndexOptions=Index vector (dialog)  Indices=1  OutputSizes=1
  Demux_AngularRates : Demux  Outputs=3
  Mux_RateSetpoints : Mux  Inputs=3
  RateIntegral_State : Subsystem  Variant=on
  RatePID_Core : Subsystem
  UnitDelay_RateIntegral : UnitDelay  InitialCondition=[0,0,0]  SampleTime=-1
  torque_yaw_filtered : Outport
  torque_pitch : Outport  Port=2
  torque_roll : Outport  Port=3
  wires:
  rate_sp_yaw_rads/1 -> Mux_RateSetpoints/3  "yaw_rate"
  ControlPower_Monitor/1(control_power) -> Cast To Single/1
  dt_rate_s/1 -> Cast To Double/1
  rate_sp_roll_rads/1 -> Mux_RateSetpoints/1  "roll_rate"
  rate_sp_pitch_rads/1 -> Mux_RateSetpoints/2  "pitch_rate"
  angular_velocity_body_rads/1 -> RatePID_Core/1(angular_rate_measured_rads)
  DSR_MC_RATE_D_Gains/1 -> RatePID_Core/8(gain_D_MC_ROLLRATE_D)
  Mux_RateSetpoints/1 -> RatePID_Core/2(angular_rate_setpoint_rads)
  torque_sp_achieved_flag/1 -> RatePID_Core/3(torque_sp_achieved)
  is_landed/1 -> RatePID_Core/4(vehicle_landed)
  unallocated_torque_from_mixer/1 -> RatePID_Core/5(mixer_unallocated_torque)
  DSR_MC_RATE_P_Gains/1 -> RatePID_Core/6(gain_P_MC_ROLLRATE_P)
  DSR_MC_RATE_I_Gains/1 -> RatePID_Core/7(gain_I_MC_ROLLRATE_I)
  DSR_IntegratorLimits/1 -> RatePID_Core/9(integral_limit_MC_RR_INT_LIM)
  angular_accel_body_rads2/1 -> RatePID_Core/11(angular_accel_filtered_rads2)
  DSR_MC_RATE_FF_Gains/1 -> RatePID_Core/12(gain_FF_MC_ROLLRATE_FF)
  UnitDelay_RateIntegral/1 -> RatePID_Core/13(rate_integral_state_prev)
  Cast To Double/1 -> ControlPower_Monitor/2(dt), RatePID_Core/10(dt_s)
  Demux_AngularRates/3 -> torque_yaw_filtered/1
  RatePID_Core/2(rate_integral_state_next) -> UnitDelay_RateIntegral/1
  RatePID_Core/1(torque_setpoint_Nm) -> Demux_AngularRates/1, ControlPower_Monitor/1(vehicle_torque_setpoint)
  Demux_AngularRates/1 -> torque_roll/1
  Demux_AngularRates/2 -> torque_pitch/1
  Cast To Single/1 -> RateIntegral_State/1(Control_Power)

== system flightControlSystem/MultiCopter Controller/Attitude_Controller ==
  q_current_wxyz : Inport
  attitude_sp_roll_rad : Inport  Port=2
  attitude_sp_pitch_rad : Inport  Port=3
  attitude_sp_yaw_rad : Inport  Port=4
  q_delta_smoothing : Inport  Port=5
  function : TriggerPort  TriggerType=function-call  VariantControl=(inherit)
  AttitudeControl : Subsystem
  Cast To Single{,1..7} (8 alike) : DataTypeConversion  OutDataTypeStr=single  SaturateOnIntegerOverflow=off  RndMeth=Floor
  DSR_MC_ATT_P_Gains : DataStoreRead  DataStoreName=PX4_Params  DataStoreElements=PX4_Params.MC_ATT_P  IndexOptions=Index vector (dialog)  Indices=1  OutputSizes=1
  DSR_MC_YAW_WEIGHT : DataStoreRead  DataStoreName=PX4_Params  DataStoreElements=PX4_Params.MC_YAW_WEIGHT  IndexOptions=Index vector (dialog)  Indices=1  OutputSizes=1
  Demux_RateSetpoints_RPY : Demux  Outputs=3
  EulerToQuaternion_Setpoint : MATLAB Function  TreatAsAtomicUnit=on
  YawSetpoint_Previous : Constant  Value=0  SampleTime=-1
  rate_sp_roll_rads : Outport
  rate_sp_pitch_rads : Outport  Port=2
  rate_sp_yaw_rads : Outport  Port=3
  q_desired_prev_wxyz : Outport  Port=4
  wires:
  EulerToQuaternion_Setpoint/1(qd) -> Cast To Single7/1
  DSR_MC_YAW_WEIGHT/1 -> Cast To Single4/1
  YawSetpoint_Previous/1 -> Cast To Single5/1
  q_current_wxyz/1 -> AttitudeControl/1(q_vehicle_attitude_wxyz)
  Cast To Single3/1 -> AttitudeControl/4(MC_ATT_P_proportional_gain)
  Cast To Single6/1 -> AttitudeControl/2(q_delta_from_prev_step)
  Cast To Single7/1 -> AttitudeControl/3(q_attitude_setpoint_wxyz)
  Cast To Single5/1 -> AttitudeControl/6(yaw_rate_sp_feedforward_rads)
  Cast To Single4/1 -> AttitudeControl/5(MC_YAW_WEIGHT_0to1)
  AttitudeControl/1(body_rate_setpoint_pqr_rads) -> Demux_RateSetpoints_RPY/1
  Cast To Single2/1 -> rate_sp_roll_rads/1
  Cast To Single/1 -> rate_sp_yaw_rads/1
  Cast To Single1/1 -> rate_sp_pitch_rads/1
  attitude_sp_pitch_rad/1 -> EulerToQuaternion_Setpoint/2(pitch)  "des_pitch"
  AttitudeControl/2(q_desired_for_next_step) -> q_desired_prev_wxyz/1
  Demux_RateSetpoints_RPY/1 -> Cast To Single2/1
  Demux_RateSetpoints_RPY/2 -> Cast To Single1/1
  Demux_RateSetpoints_RPY/3 -> Cast To Single/1
  DSR_MC_ATT_P_Gains/1 -> Cast To Single3/1
  q_delta_smoothing/1 -> Cast To Single6/1
  attitude_sp_yaw_rad/1 -> EulerToQuaternion_Setpoint/3(yaw)  "des_yaw"
  attitude_sp_roll_rad/1 -> EulerToQuaternion_Setpoint/1(roll)  "des_roll"

== system flightControlSystem/MultiCopter Controller/Position & Altitude controller ==
  position_setpoint_NED_m : Inport
  vehicle_position_NED_m : Inport  Port=2
  vehicle_velocity_NED_ms : Inport  Port=3
  velocity_setpoint_NED_ms : Inport  Port=4
  accel_setpoint_NED_ms2 : Inport  Port=5
  dt_position_s : Inport  Port=6
  accel_filtered_NED_ms2 : Inport  Port=7
  yaw_setpoint_rad : Inport  Port=8
  function : TriggerPort  TriggerType=function-call  VariantControl=(inherit)
  Cast To Double : DataTypeConversion  OutDataTypeStr=double  SaturateOnIntegerOverflow=off  RndMeth=Floor
  Cast To Double1 : DataTypeConversion  OutDataTypeStr=double  SaturateOnIntegerOverflow=off  RndMeth=Floor
  Cast To Double2 : DataTypeConversion  OutDataTypeStr=double  SaturateOnIntegerOverflow=off  RndMeth=Floor
  Position controller : Subsystem
  Terminator3 : Terminator
  attitude_sp_roll_rad : Outport
  attitude_sp_pitch_rad : Outport  Port=2
  attitude_sp_yaw_rad : Outport  Port=3
  thrust_setpoint_normalized : Outport  Port=4
  wires:
  vehicle_velocity_NED_ms/1 -> Cast To Double1/1
  position_setpoint_NED_m/1 -> Position controller/1(position_setpoint_NED_m)
  vehicle_position_NED_m/1 -> Cast To Double/1
  accel_filtered_NED_ms2/1 -> Cast To Double2/1
  Cast To Double/1 -> Position controller/2(vehicle_local_position_m)
  Cast To Double1/1 -> Position controller/3(vehicle_velocity_NED_ms)
  Position controller/4(thrust_normalized_0to1) -> thrust_setpoint_normalized/1
  Position controller/3(attitude_sp_roll_rad) -> attitude_sp_roll_rad/1
  Position controller/2(attitude_sp_pitch_rad) -> attitude_sp_pitch_rad/1
  Position controller/1(yaw_sp_passthrough_rad) -> attitude_sp_yaw_rad/1
  dt_position_s/1 -> Position controller/7(dt_s)
  Cast To Double2/1 -> Position controller/8(vehicle_accel_filtered_ms2)
  yaw_setpoint_rad/1 -> Position controller/4(yaw_setpoint_rad)
  velocity_setpoint_NED_ms/1 -> Position controller/5(velocity_setpoint_NED_ms)
  accel_setpoint_NED_ms2/1 -> Position controller/6(accel_setpoint_feedforward_ms2)
  Position controller/5(hover_thrust_adaptive) -> Terminator3/1

== system flightControlSystem/MultiCopter Controller/Quaternion Validity Check ==
  In1 : Inport
  Constant : Constant  Value=[1 0 0 0]  SampleTime=-1
  Quaternion Norm : sharedutil/Quaternion Norm  aMode=aMode
  Switch : Switch  Criteria=u2 > Threshold  SaturateOnIntegerOverflow=off  InputSameDT=off
  Valid quat : Outport
  wires:
  In1/1 -> Quaternion Norm/1, Switch/1
  Quaternion Norm/1 -> Switch/2
  Switch/1 -> Valid quat/1
  Constant/1 -> Switch/3

== system flightControlSystem/MultiCopter Controller/Quaternion Validity Check1 ==
  In1 : Inport
  Constant : Constant  Value=[1 0 0 0]  SampleTime=-1
  Quaternion Norm : sharedutil/Quaternion Norm  aMode=aMode
  Switch : Switch  Criteria=u2 > Threshold  SaturateOnIntegerOverflow=off  InputSameDT=off
  Valid quat : Outport
  wires:
  In1/1 -> Quaternion Norm/1, Switch/1
  Quaternion Norm/1 -> Switch/2
  Switch/1 -> Valid quat/1
  Constant/1 -> Switch/3

== system flightControlSystem/ParamUpdate/HW_ParamUpdate ==
  FirstRun_Pulse : UnitDelay  InitialCondition=true
  FirstRun_Zero : Constant  Value=0  OutDataTypeStr=boolean  SampleTime=1
  IsNewParamUpdate : simulink/Logic and Bit Operations/Compare To Constant  relop===  const=0  OutDataTypeStr=boolean
  ReadParams_Enable : Logic  Operator=OR  AllPortsSameDT=off  OutDataTypeStr=boolean
  ReadParams_OnUpdate : Subsystem
  Term_ParamUpdateMsg : Terminator
  uORB_ParameterUpdate : px4uORBlib/PX4 uORB Read  uORBMsg=ParameterUpdate  uORBTopicName=parameter_update  SubscribeNonZeroInstance=off  selectInstanceNum=1  SampleTime=1  isSingleTopicMsg=on  BlockingMode=off  BlockTimeout=1e-3
  wires:
  uORB_ParameterUpdate/1 -> IsNewParamUpdate/1
  uORB_ParameterUpdate/2 -> Term_ParamUpdateMsg/1
  FirstRun_Zero/1 -> FirstRun_Pulse/1
  IsNewParamUpdate/1 -> ReadParams_Enable/1
  FirstRun_Pulse/1 -> ReadParams_Enable/2
  ReadParams_Enable/1 -> ReadParams_OnUpdate/Enable

== system flightControlSystem/ParamUpdate/SimParamUpdate ==
  ParamConstants : Constant  Value=PX4_Params_Default  OutDataTypeStr=Bus: PX4_Params_Bus  SampleTime=1
  Write_PX4_Params : DataStoreWrite  DataStoreName=PX4_Params  IndexOptions=Index vector (dialog)  Indices=1  OutputSizes=1
  wires:
  ParamConstants/1 -> Write_PX4_Params/1

== system flightControlSystem/SetpointManager/Set target Position ==
  vehicle_position_NED_m : Inport
  Landing Logic : Subsystem
  Logger : Subsystem
  RC Failsafe Signal : Subsystem
  Rate Transition1 : RateTransition  OutPortSampleTime=1/10
  Setpoints Selector : Subsystem
  Setpoints from Perception Module : Subsystem
  velocity_setpoint_NED_ms : Outport
  accel_setpoint_NED_ms2 : Outport  Port=2
  position_setpoint_NED_m : Outport  Port=3
  wires:
  Setpoints Selector/3(des_acc) -> accel_setpoint_NED_ms2/1, Logger/3(DesiredAcceleration)
  RC Failsafe Signal/1(Land_Trigger) -> Setpoints Selector/4(LandTrigger), Landing Logic/2(land_trigger)
  vehicle_position_NED_m/1 -> Rate Transition1/1
  Landing Logic/1(pos_sp) -> Setpoints Selector/1(Land_Pos)
  Landing Logic/3(acc_sp) -> Setpoints Selector/3(Land_Acc)
  Setpoints Selector/1(des_pos) -> Logger/1(DesiredPosition), position_setpoint_NED_m/1
  Setpoints Selector/2(des_vel) -> Logger/2(DesiredVelocity), velocity_setpoint_NED_ms/1
  Landing Logic/2(vel_sp) -> Setpoints Selector/2(Land_Vel)
  Rate Transition1/1 -> Logger/4(States), Setpoints from Perception Module/1(CurrentPosition), Landing Logic/1(Current_Pos)
  Setpoints from Perception Module/1(des Position) -> Setpoints Selector/5(Des_Pos)
  Setpoints from Perception Module/2(desired Velocity) -> Setpoints Selector/6(Des_Vel)
  Setpoints from Perception Module/3(desired Acceleration) -> Setpoints Selector/7(Des_Acc)

== system flightControlSystem/SetpointManager/Simulation Set target Position ==
  raw_position_command_NED : Inport
  vehicle_position_NED_m : Inport  Port=2
  Bus to Vector : BusToVector
  Constant : Constant  Value=0  SampleTime=-1
  Constant1 : Constant  SampleTime=-1
  Constant2 : Constant  Value=0  SampleTime=-1
  Demux : Demux  Outputs=11
  Landing Logic : Subsystem
  Mux : Mux
  Mux1 : Mux  Inputs=3
  Mux2 : Mux  Inputs=3
  Setpoints Selector : Subsystem
  Switch1 : Switch  Criteria=u2 ~= 0  SaturateOnIntegerOverflow=off  InputSameDT=off
  Terminator3 : Terminator
  position_setpoint_NED_m : Outport
  velocity_setpoint_NED_ms : Outport  Port=2
  accel_setpoint_NED_ms2 : Outport  Port=3
  wires:
  Bus to Vector/1 -> Demux/1
  Constant2/1 -> Switch1/2
  raw_position_command_NED/1 -> Bus to Vector/1
  Constant1/1 -> Switch1/1
  Constant/1 -> Switch1/3
  Switch1/1 -> Setpoints Selector/4(LandTrigger), Landing Logic/2(land_trigger)
  Demux/1 -> Mux/1
  Demux/2 -> Mux/2
  Demux/3 -> Mux/3
  Demux/4 -> Mux/4
  Demux/5 -> Mux1/1
  Demux/6 -> Mux1/2
  Demux/7 -> Mux1/3
  Demux/8 -> Mux2/1
  Demux/9 -> Mux2/2
  Demux/10 -> Mux2/3
  Demux/11 -> Terminator3/1
  Setpoints Selector/1(des_pos) -> position_setpoint_NED_m/1
  vehicle_position_NED_m/1 -> Landing Logic/1(Current_Pos)
  Landing Logic/1(pos_sp) -> Setpoints Selector/1(Land_Pos)
  Landing Logic/2(vel_sp) -> Setpoints Selector/2(Land_Vel)
  Landing Logic/3(acc_sp) -> Setpoints Selector/3(Land_Acc)
  Mux/1 -> Setpoints Selector/5(Des_Pos)
  Mux1/1 -> Setpoints Selector/6(Des_Vel)
  Mux2/1 -> Setpoints Selector/7(Des_Acc)
  Setpoints Selector/2(des_vel) -> velocity_setpoint_NED_ms/1
  Setpoints Selector/3(des_acc) -> accel_setpoint_NED_ms2/1

== system flightControlSystem/Actuator Commands/Actuator Commands/Using PX4 Mixers  ==
  note: Note:
      | 1. All the values are in the drone body FRD frame.
      | 2. Positive z is downwards in the FRD frame, so 'thrust_z' is negative.
  tau_Thrust : Inport
  tau_Pitch : Inport  Port=2
  tau_Roll : Inport  Port=3
  tau_yaw : Inport  Port=4
  Bus Selector : BusSelector  OutputSignals=voltage_v,current_a,current_average_a,discharged_mah,scale
  Cast To Single{2..5} (4 alike) : DataTypeConversion  OutDataTypeStr=single  SaturateOnIntegerOverflow=off  RndMeth=Floor
  Compare To Constant : simulink/Logic and Bit Operations/Compare To Constant  relop=~=  const=0  OutDataTypeStr=boolean
  PX4 ULog : px4Utilslib/PX4 ULog  Commented=on  uORBMsg=BatteryLogging
  PX4 Write Thrust & Torque Setpoint : px4Utilslib/PX4 Write Thrust & Torque Setpoint
  PX4 uORB Read5 : px4uORBlib/PX4 uORB Read  uORBMsg=BatteryStatus  uORBTopicName=battery_status  SubscribeNonZeroInstance=off  selectInstanceNum=1  SampleTime=-1  isSingleTopicMsg=on  BlockingMode=off  BlockTimeout=1e-3
  Product : Product
  Product1 : Product
  Saturation : Saturate  UpperLimit=1  LowerLimit=-1
  Saturation1 : Saturate  UpperLimit=1  LowerLimit=-1
  Switch : Switch  Criteria=u2 > Threshold  SaturateOnIntegerOverflow=off  InputSameDT=off
  Switch1 : Switch  Criteria=u2 > Threshold  SaturateOnIntegerOverflow=off  InputSameDT=off
  Terminator7 : Terminator
  Vector Concatenate1 : Concatenate  NumInputs=3
  wires:
  PX4 uORB Read5/1 -> Terminator7/1
  PX4 uORB Read5/2 -> Bus Selector/1
  Bus Selector/2 -> Cast To Single3/1  "<current_a>"
  tau_yaw/1 -> Vector Concatenate1/3
  tau_Roll/1 -> Vector Concatenate1/1
  tau_Pitch/1 -> Vector Concatenate1/2
  Bus Selector/1 -> Cast To Single2/1  "<voltage_v>"
  Vector Concatenate1/1 -> Switch1/3, Product1/1
  Bus Selector/3 -> Cast To Single4/1  "<current_average_a>"
  Bus Selector/4 -> Cast To Single5/1  "<discharged_mah>"
  Bus Selector/5 -> Compare To Constant/1, Product/2, Product1/2  "<scale>"
  tau_Thrust/1 -> Switch/3, Product/1
  Cast To Single2/1 -> PX4 ULog/1
  Cast To Single3/1 -> PX4 ULog/2
  Cast To Single4/1 -> PX4 ULog/3
  Cast To Single5/1 -> PX4 ULog/4
  Compare To Constant/1 -> Switch1/2, Switch/2
  Product/1 -> Switch/1
  Product1/1 -> Switch1/1
  Switch/1 -> Saturation1/1
  Switch1/1 -> Saturation/1
  Saturation1/1 -> PX4 Write Thrust & Torque Setpoint/1
  Saturation/1 -> PX4 Write Thrust & Torque Setpoint/2

== system flightControlSystem/Actuator Commands/Simulation Actuator Commands/Mixer ==
  tau_Thrust : Inport
  tau_yaw : Inport  Port=2
  tau_Pitch : Inport  Port=3
  tau_Roll : Inport  Port=4
  Battery_Scaling : Subsystem
  Bus Creator1 : BusCreator  Inputs=8  OutDataTypeStr=Bus: setPWMInput
  Demux : Demux  Outputs=3
  Demux2 : Demux  Outputs=8
  MATLAB Function : MATLAB Function  TreatAsAtomicUnit=on
  Saturation : Saturate  UpperLimit=1  LowerLimit=0
  String Constant : StringConstant  String=frameType
  Terminator : Terminator
  Terminator1 : Terminator
  Vector Concatenate1 : Concatenate  NumInputs=3
  PWM_Input : Outport
  wires:
  Demux/1 -> Terminator/1
  Demux/2 -> Terminator1/1
  Demux/3 -> Battery_Scaling/1(In1)
  tau_Thrust/1 -> Demux/1
  tau_yaw/1 -> Vector Concatenate1/3
  Vector Concatenate1/1 -> Battery_Scaling/2(In2)
  tau_Roll/1 -> Vector Concatenate1/1
  tau_Pitch/1 -> Vector Concatenate1/2
  String Constant/1 -> MATLAB Function/1(frameType)
  Battery_Scaling/4(yaw) -> MATLAB Function/5(yaw)
  Battery_Scaling/3(roll) -> MATLAB Function/4(roll)
  Battery_Scaling/2(pitch) -> MATLAB Function/3(pitch)
  Battery_Scaling/1(thrust_setpoint) -> MATLAB Function/2(thrust)
  Demux2/3 -> Bus Creator1/3  "M3"
  MATLAB Function/1(rotor_cmd) -> Saturation/1
  Demux2/8 -> Bus Creator1/8  "M8"
  Demux2/1 -> Bus Creator1/1  "M1"
  Demux2/2 -> Bus Creator1/2  "M2"
  Demux2/4 -> Bus Creator1/4  "M4"
  Demux2/5 -> Bus Creator1/5  "M5"
  Demux2/6 -> Bus Creator1/6  "M6"
  Demux2/7 -> Bus Creator1/7  "M7"
  Bus Creator1/1 -> PWM_Input/1
  Saturation/1 -> Demux2/1

== system flightControlSystem/Estimator/Simulation Estimator/Quaternion Validity Check ==
  Current_Attitude : Inport
  Constant : Constant  Value=[1 0 0 0]  SampleTime=-1
  Quaternion Norm : sharedutil/Quaternion Norm  aMode=aMode
  Switch : Switch  Criteria=u2 > Threshold  SaturateOnIntegerOverflow=off  InputSameDT=off
  Valid quat : Outport
  wires:
  Current_Attitude/1 -> Quaternion Norm/1, Switch/1
  Quaternion Norm/1 -> Switch/2
  Switch/1 -> Valid quat/1
  Constant/1 -> Switch/3

== system flightControlSystem/MultiCopter Controller/Angular Rate Control/RateIntegral_State ==
  note: 1) Add Subsystem or Model blocks as valid variant choices.
      | 2) You cannot connect blocks at this level. At simulation, connectivity is automatically
      | determined, based on the active variant and port name matching.
  Control_Power : Inport
  Set target Position : Subsystem  VariantControl=Simulation == false
  Simulation Set target Position : Subsystem  VariantControl=Simulation == true
